simulink model "Hybrid_OpAmp_Integral"
settings: Solver=ode23t  StopTime=0.001  RelTol=1e-5  AbsTol=1e-6
settings Model: Creator=Senior Analog IC & SET Device Design Engineer  LastModifiedBy=Antigravity MATLAB Automation

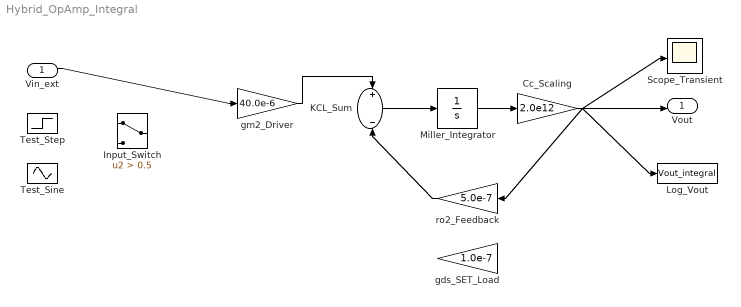
== system Hybrid_OpAmp_Integral ==
  Vin_ext : Inport  Port=1
  Test_Step : Step  Time=0.0001  Before=0  After=0.01
  Test_Sine : Sin  Amplitude=0.005  Frequency=6283.1853
  Input_Switch : Switch  Criteria=u2 > Threshold  Threshold=0.5
  gm2_Driver : Gain  Gain=40.0e-6
  KCL_Sum : Sum  Inputs=+-
  Miller_Integrator : Integrator  InitialCondition=0.4  LimitOutput=on  UpperSaturationLimit=0.75  LowerSaturationLimit=0.05
  Cc_Scaling : Gain  Gain=2.0e12
  ro2_Feedback : Gain  Gain=5.0e-7  Orientation=left
  gds_SET_Load : Gain  Gain=1.0e-7  Orientation=left
  Vout : Outport  Port=1
  Scope_Transient : Scope
  Log_Vout : ToWorkspace  VariableName=Vout_integral  SaveFormat=Array
  wires:
  Vin_ext/1 -> gm2_Driver/1
  gm2_Driver/1 -> KCL_Sum/1
  KCL_Sum/1 -> Miller_Integrator/1
  Miller_Integrator/1 -> Cc_Scaling/1
  Cc_Scaling/1 -> Vout/1
  Cc_Scaling/1 -> Scope_Transient/1
  Cc_Scaling/1 -> Log_Vout/1
  Cc_Scaling/1 -> ro2_Feedback/1
  ro2_Feedback/1 -> KCL_Sum/2
